simulink library "single_phase_three_levels_PWM_modulator"  (R2025b)
settings: Solver=VariableStepAuto  StartTime=0.0  StopTime=10.0  RelTol=1e-3
undefined symbols (not defined in the file): dead_time_INV, fPWM_INV, tc
libraries: single_phase_pwm_modulator x1
settings Model: Creator=dbagn  LastModifiedBy=dbagn

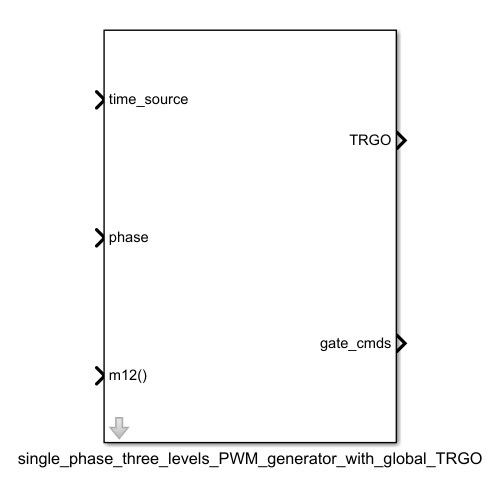
[thumbnail: Simulink's stored preview of the top-level diagram]
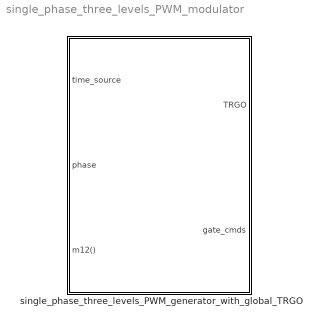
== system single_phase_three_levels_PWM_modulator ==
  single_phase_three_levels_PWM_generator_with_global_TRGO : Subsystem  mask{f=fPWM_INV, m_up=1, m_low=-1, dead_time=dead_time_INV, pos_cmd_gate=15, neg_cmd_gate=-10, polarity=1, tc=tc, double_sampling=1}
      mask prompts: f "Frequency (Hz)"; m_up "Max Input Modulation Value"; m_low "Min Input Modulation Value"; dead_time "Dead Time (s)"; pos_cmd_gate "Positive Gate Voltage (V)"; neg_cmd_gate "Negative Gate Voltage (V)"; polarity "Polarity (pu)"; tc "Sampling time"; double_sampling "double TRGO update"

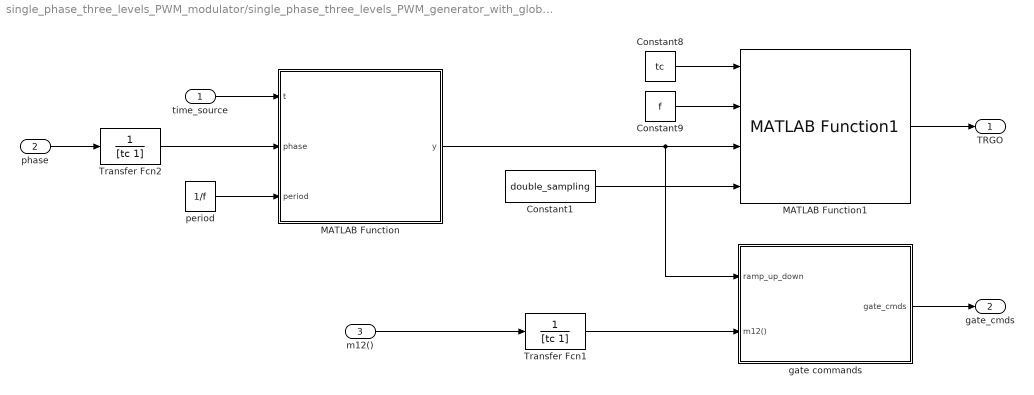
== system single_phase_three_levels_PWM_modulator/single_phase_three_levels_PWM_generator_with_global_TRGO ==
  time_source : Inport
  phase : Inport  Port=2
  m12() : Inport  Port=3
  Constant1 : Constant  Value=double_sampling
  Constant8 : Constant  Value=tc
  Constant9 : Constant  Value=f
  MATLAB Function : MATLAB Function  TreatAsAtomicUnit=on  SystemSampleTime=tc
  MATLAB Function1 : single_phase_pwm_modulator/Single phase two level PWM generator with global TRGO/MATLAB Function1  SystemSampleTime=tc  VariantActivationTime=update diagram  EmptyChoice=off  PassThrough=off  PassThroughVariantControl=(default)  EmptyChoiceVariantControl=(default)  AllowFlexibleInterface=on  Latency=0  AutoFrameSizeCalculation=off
  Transfer Fcn1 : TransferFcn  Denominator=[tc 1]
  Transfer Fcn2 : TransferFcn  Denominator=[tc 1]
  gate commands : Subsystem
  period : Constant  Value=1/f
  TRGO : Outport
  gate_cmds : Outport  Port=2
  wires:
  period/1 -> MATLAB Function/3(period)
  phase/1 -> Transfer Fcn2/1
  MATLAB Function/1(y) -> gate commands/1(ramp_up_down), MATLAB Function1/3
  MATLAB Function1/1 -> TRGO/1
  Constant8/1 -> MATLAB Function1/1
  Constant9/1 -> MATLAB Function1/2
  m12()/1 -> Transfer Fcn1/1
  gate commands/1(gate_cmds) -> gate_cmds/1
  time_source/1 -> MATLAB Function/1(t)
  Constant1/1 -> MATLAB Function1/4
  Transfer Fcn2/1 -> MATLAB Function/2(phase)
  Transfer Fcn1/1 -> gate commands/2(m12())

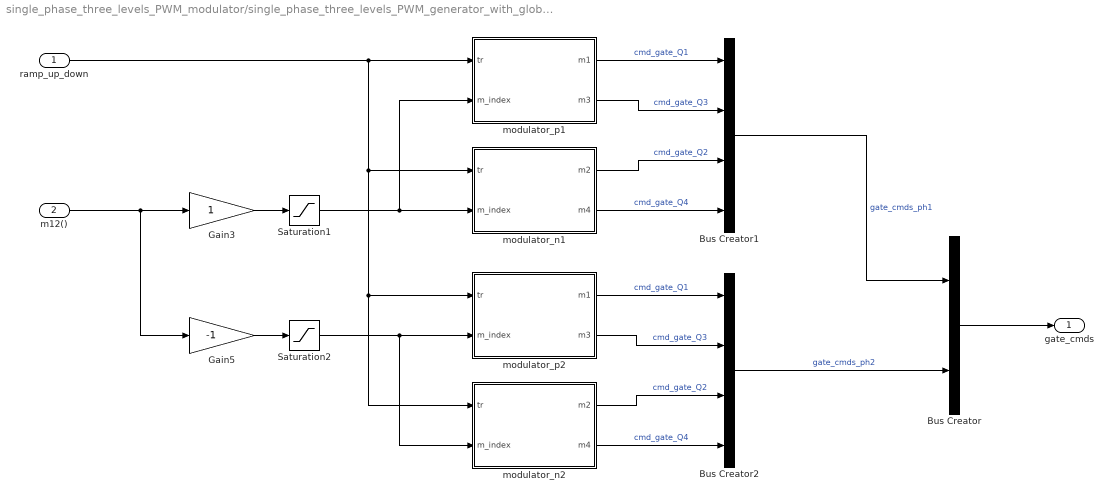
== system single_phase_three_levels_PWM_modulator/single_phase_three_levels_PWM_generator_with_global_TRGO/gate commands ==
  ramp_up_down : Inport
  m12() : Inport  Port=2
  Bus Creator : BusCreator  Inputs=2
  Bus Creator1 : BusCreator  Inputs=4
  Bus Creator2 : BusCreator  Inputs=4
  Gain3 : Gain
  Gain5 : Gain  Gain=-1
  Saturation1 : Saturate  UpperLimit=m_up  LowerLimit=m_low
  Saturation2 : Saturate  UpperLimit=m_up  LowerLimit=m_low
  modulator_n1 : Subsystem
  modulator_n2 : Subsystem
  modulator_p1 : Subsystem
  modulator_p2 : Subsystem
  gate_cmds : Outport
  wires:
  Saturation2/1 -> modulator_n2/2(m_index), modulator_p2/2(m_index)
  ramp_up_down/1 -> modulator_p1/1(tr), modulator_n1/1(tr), modulator_p2/1(tr), modulator_n2/1(tr)
  modulator_p2/1(m1) -> Bus Creator2/1  "cmd_gate_Q1"
  modulator_p2/2(m3) -> Bus Creator2/2  "cmd_gate_Q3"
  modulator_n2/1(m2) -> Bus Creator2/3  "cmd_gate_Q2"
  modulator_n2/2(m4) -> Bus Creator2/4  "cmd_gate_Q4"
  Bus Creator2/1 -> Bus Creator/2  "gate_cmds_ph2"
  Bus Creator1/1 -> Bus Creator/1  "gate_cmds_ph1"
  modulator_n1/2(m4) -> Bus Creator1/4  "cmd_gate_Q4"
  modulator_n1/1(m2) -> Bus Creator1/3  "cmd_gate_Q2"
  modulator_p1/2(m3) -> Bus Creator1/2  "cmd_gate_Q3"
  modulator_p1/1(m1) -> Bus Creator1/1  "cmd_gate_Q1"
  Gain3/1 -> Saturation1/1
  Bus Creator/1 -> gate_cmds/1
  Gain5/1 -> Saturation2/1
  m12()/1 -> Gain5/1, Gain3/1
  Saturation1/1 -> modulator_n1/2(m_index), modulator_p1/2(m_index)

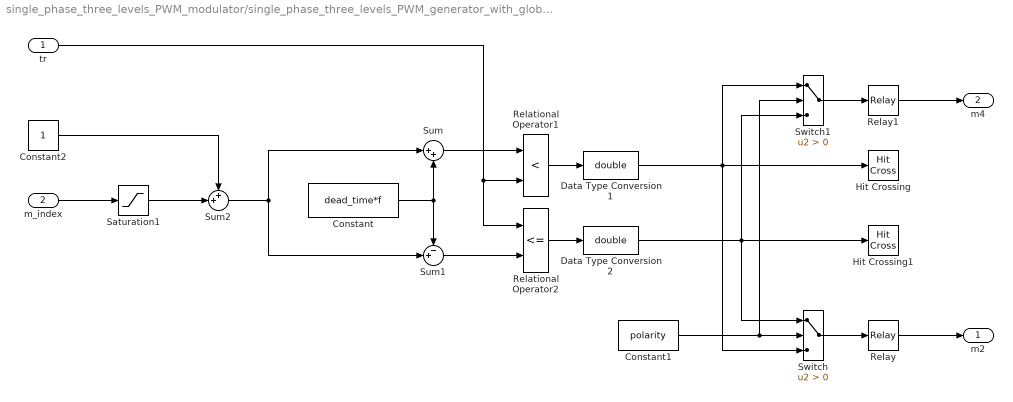
== system single_phase_three_levels_PWM_modulator/single_phase_three_levels_PWM_generator_with_global_TRGO/gate commands/modulator_n1 ==
  tr : Inport
  m_index : Inport  Port=2
  Constant : Constant  Value=dead_time*f
  Constant1 : Constant  Value=polarity
  Constant2 : Constant
  Data Type Conversion1 : DataTypeConversion  OutDataTypeStr=double
  Data Type Conversion2 : DataTypeConversion  OutDataTypeStr=double
  Hit Crossing : HitCross  ShowOutputPort=off
  Hit Crossing1 : HitCross  ShowOutputPort=off
  Relational Operator1 : RelationalOperator  Operator=<  InputSameDT=off
  Relational Operator2 : RelationalOperator  Operator=<=  InputSameDT=off
  Relay : Relay  OnOutputValue=pos_cmd_gate  OffOutputValue=neg_cmd_gate
  Relay1 : Relay  OnOutputValue=pos_cmd_gate  OffOutputValue=neg_cmd_gate
  Saturation1 : Saturate  UpperLimit=0  LowerLimit=m_low
  Sum : Sum  Inputs=|++  SaturateOnIntegerOverflow=on
  Sum1 : Sum  Inputs=-+|  SaturateOnIntegerOverflow=on
  Sum2 : Sum  Inputs=++|  SaturateOnIntegerOverflow=on
  Switch : Switch  Criteria=u2 > Threshold  SaturateOnIntegerOverflow=off  InputSameDT=off
  Switch1 : Switch  Criteria=u2 > Threshold  SaturateOnIntegerOverflow=off  InputSameDT=off
  m2 : Outport
  m4 : Outport  Port=2
  wires:
  Constant2/1 -> Sum2/1
  Sum2/1 -> Sum/1, Sum1/2
  Saturation1/1 -> Sum2/2
  m_index/1 -> Saturation1/1
  Relational Operator2/1 -> Data Type Conversion2/1
  Relational Operator1/1 -> Data Type Conversion1/1
  Data Type Conversion1/1 -> Hit Crossing/1, Switch/3, Switch1/1
  Sum1/1 -> Relational Operator2/2
  Constant1/1 -> Switch1/2, Switch/2
  Data Type Conversion2/1 -> Switch/1, Switch1/3, Hit Crossing1/1
  Switch/1 -> Relay/1
  Constant/1 -> Sum/2, Sum1/1
  Sum/1 -> Relational Operator1/1
  tr/1 -> Relational Operator2/1, Relational Operator1/2
  Switch1/1 -> Relay1/1
  Relay/1 -> m2/1
  Relay1/1 -> m4/1

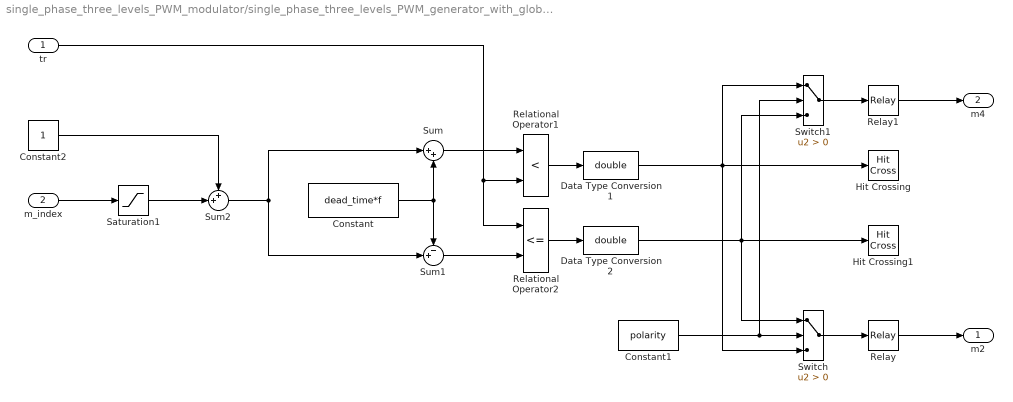
== system single_phase_three_levels_PWM_modulator/single_phase_three_levels_PWM_generator_with_global_TRGO/gate commands/modulator_n2 ==
  tr : Inport
  m_index : Inport  Port=2
  Constant : Constant  Value=dead_time*f
  Constant1 : Constant  Value=polarity
  Constant2 : Constant
  Data Type Conversion1 : DataTypeConversion  OutDataTypeStr=double
  Data Type Conversion2 : DataTypeConversion  OutDataTypeStr=double
  Hit Crossing : HitCross  ShowOutputPort=off
  Hit Crossing1 : HitCross  ShowOutputPort=off
  Relational Operator1 : RelationalOperator  Operator=<  InputSameDT=off
  Relational Operator2 : RelationalOperator  Operator=<=  InputSameDT=off
  Relay : Relay  OnOutputValue=pos_cmd_gate  OffOutputValue=neg_cmd_gate
  Relay1 : Relay  OnOutputValue=pos_cmd_gate  OffOutputValue=neg_cmd_gate
  Saturation1 : Saturate  UpperLimit=0  LowerLimit=m_low
  Sum : Sum  Inputs=|++  SaturateOnIntegerOverflow=on
  Sum1 : Sum  Inputs=-+|  SaturateOnIntegerOverflow=on
  Sum2 : Sum  Inputs=++|  SaturateOnIntegerOverflow=on
  Switch : Switch  Criteria=u2 > Threshold  SaturateOnIntegerOverflow=off  InputSameDT=off
  Switch1 : Switch  Criteria=u2 > Threshold  SaturateOnIntegerOverflow=off  InputSameDT=off
  m2 : Outport
  m4 : Outport  Port=2
  wires:
  Relay1/1 -> m4/1
  Relay/1 -> m2/1
  Switch1/1 -> Relay1/1
  tr/1 -> Relational Operator1/2, Relational Operator2/1
  Sum/1 -> Relational Operator1/1
  Constant/1 -> Sum1/1, Sum/2
  Switch/1 -> Relay/1
  Data Type Conversion2/1 -> Hit Crossing1/1, Switch1/3, Switch/1
  Constant1/1 -> Switch/2, Switch1/2
  Sum1/1 -> Relational Operator2/2
  Data Type Conversion1/1 -> Switch1/1, Switch/3, Hit Crossing/1
  Relational Operator1/1 -> Data Type Conversion1/1
  Relational Operator2/1 -> Data Type Conversion2/1
  m_index/1 -> Saturation1/1
  Saturation1/1 -> Sum2/2
  Sum2/1 -> Sum1/2, Sum/1
  Constant2/1 -> Sum2/1

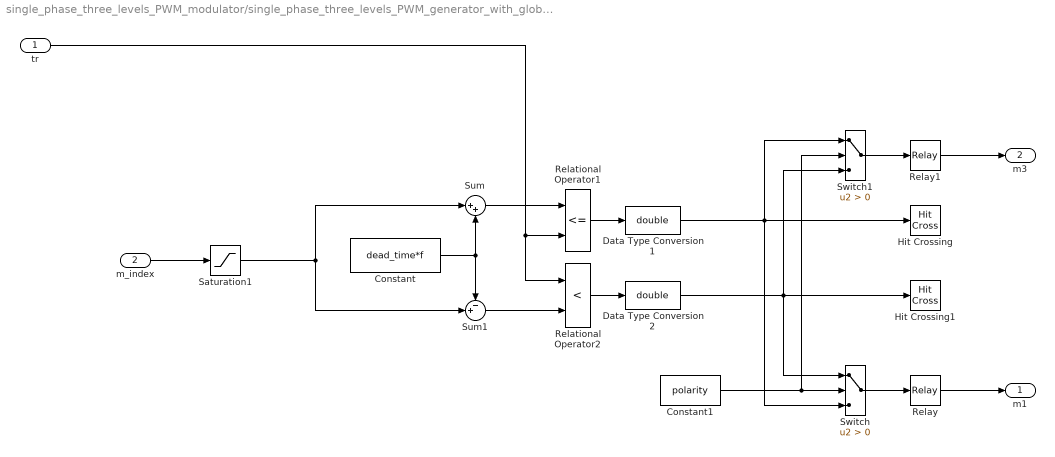
== system single_phase_three_levels_PWM_modulator/single_phase_three_levels_PWM_generator_with_global_TRGO/gate commands/modulator_p1 ==
  tr : Inport
  m_index : Inport  Port=2
  Constant : Constant  Value=dead_time*f
  Constant1 : Constant  Value=polarity
  Data Type Conversion1 : DataTypeConversion  OutDataTypeStr=double
  Data Type Conversion2 : DataTypeConversion  OutDataTypeStr=double
  Hit Crossing : HitCross  ShowOutputPort=off
  Hit Crossing1 : HitCross  ShowOutputPort=off
  Relational Operator1 : RelationalOperator  Operator=<=  InputSameDT=off
  Relational Operator2 : RelationalOperator  Operator=<  InputSameDT=off
  Relay : Relay  OnSwitchValue=2*eps  OnOutputValue=pos_cmd_gate  OffOutputValue=neg_cmd_gate
  Relay1 : Relay  OnOutputValue=pos_cmd_gate  OffOutputValue=neg_cmd_gate
  Saturation1 : Saturate  UpperLimit=m_up  LowerLimit=0
  Sum : Sum  Inputs=|++  SaturateOnIntegerOverflow=on
  Sum1 : Sum  Inputs=-+|  SaturateOnIntegerOverflow=on
  Switch : Switch  Criteria=u2 > Threshold  SaturateOnIntegerOverflow=off  InputSameDT=off
  Switch1 : Switch  Criteria=u2 > Threshold  SaturateOnIntegerOverflow=off  InputSameDT=off
  m1 : Outport
  m3 : Outport  Port=2
  wires:
  Relay1/1 -> m3/1
  Relay/1 -> m1/1
  Switch1/1 -> Relay1/1
  tr/1 -> Relational Operator1/2, Relational Operator2/1
  Sum/1 -> Relational Operator1/1
  Constant/1 -> Sum1/1, Sum/2
  Switch/1 -> Relay/1
  Data Type Conversion2/1 -> Hit Crossing1/1, Switch1/3, Switch/1
  Constant1/1 -> Switch/2, Switch1/2
  Saturation1/1 -> Sum1/2, Sum/1
  Sum1/1 -> Relational Operator2/2
  Data Type Conversion1/1 -> Switch1/1, Switch/3, Hit Crossing/1
  Relational Operator1/1 -> Data Type Conversion1/1
  Relational Operator2/1 -> Data Type Conversion2/1
  m_index/1 -> Saturation1/1

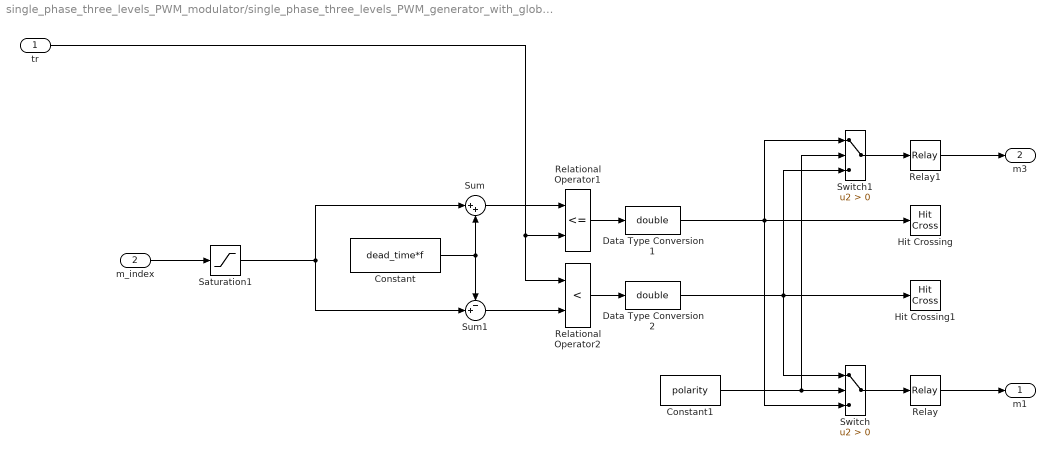
== system single_phase_three_levels_PWM_modulator/single_phase_three_levels_PWM_generator_with_global_TRGO/gate commands/modulator_p2 ==
  tr : Inport
  m_index : Inport  Port=2
  Constant : Constant  Value=dead_time*f
  Constant1 : Constant  Value=polarity
  Data Type Conversion1 : DataTypeConversion  OutDataTypeStr=double
  Data Type Conversion2 : DataTypeConversion  OutDataTypeStr=double
  Hit Crossing : HitCross  ShowOutputPort=off
  Hit Crossing1 : HitCross  ShowOutputPort=off
  Relational Operator1 : RelationalOperator  Operator=<=  InputSameDT=off
  Relational Operator2 : RelationalOperator  Operator=<  InputSameDT=off
  Relay : Relay  OnSwitchValue=2*eps  OnOutputValue=pos_cmd_gate  OffOutputValue=neg_cmd_gate
  Relay1 : Relay  OnOutputValue=pos_cmd_gate  OffOutputValue=neg_cmd_gate
  Saturation1 : Saturate  UpperLimit=m_up  LowerLimit=0
  Sum : Sum  Inputs=|++  SaturateOnIntegerOverflow=on
  Sum1 : Sum  Inputs=-+|  SaturateOnIntegerOverflow=on
  Switch : Switch  Criteria=u2 > Threshold  SaturateOnIntegerOverflow=off  InputSameDT=off
  Switch1 : Switch  Criteria=u2 > Threshold  SaturateOnIntegerOverflow=off  InputSameDT=off
  m1 : Outport
  m3 : Outport  Port=2
  wires:
  m_index/1 -> Saturation1/1
  Relational Operator2/1 -> Data Type Conversion2/1
  Relational Operator1/1 -> Data Type Conversion1/1
  Data Type Conversion1/1 -> Hit Crossing/1, Switch/3, Switch1/1
  Sum1/1 -> Relational Operator2/2
  Saturation1/1 -> Sum/1, Sum1/2
  Constant1/1 -> Switch1/2, Switch/2
  Data Type Conversion2/1 -> Switch/1, Switch1/3, Hit Crossing1/1
  Switch/1 -> Relay/1
  Constant/1 -> Sum/2, Sum1/1
  Sum/1 -> Relational Operator1/1
  tr/1 -> Relational Operator2/1, Relational Operator1/2
  Switch1/1 -> Relay1/1
  Relay/1 -> m1/1
  Relay1/1 -> m3/1

== matlab function single_phase_three_levels_PWM_modulator/single_phase_three_levels_PWM_generator_with_global_TRGO/MATLAB Function ==
  data: t input; y output; phase input; period input
function y = ramp_up_down(t,phase,period)
x = sin(2*pi/period*t - phase -pi/2);
y = asin(x)/pi + 1/2;
